simulink model "knee_assist_rev27"  (R2026b)
settings: Solver=ode1  StartTime=0  StopTime=ka_sl.t_end  FixedStep=ka_sl.dt
PostLoadFcn:
  | addpath(fileparts(get_param('knee_assist_rev27', 'FileName')));
InitFcn:
  | addpath(fileparts(get_param('knee_assist_rev27', 'FileName'))); clear sl_ka_logic sl_ka_plant; if ~(exist('ka_sl','var') && exist('ka_p','var') && exist('ka_cfg','var')), ka_simulink_setup; end
undefined symbols (not defined in the file or in its folder): ka_sl, sl_ka_logic, sl_ka_plant
settings Model: Creator=SDP II team  LastModifiedBy=SDP II team
settings DataIOCC: SaveOutput=off  SaveTime=off

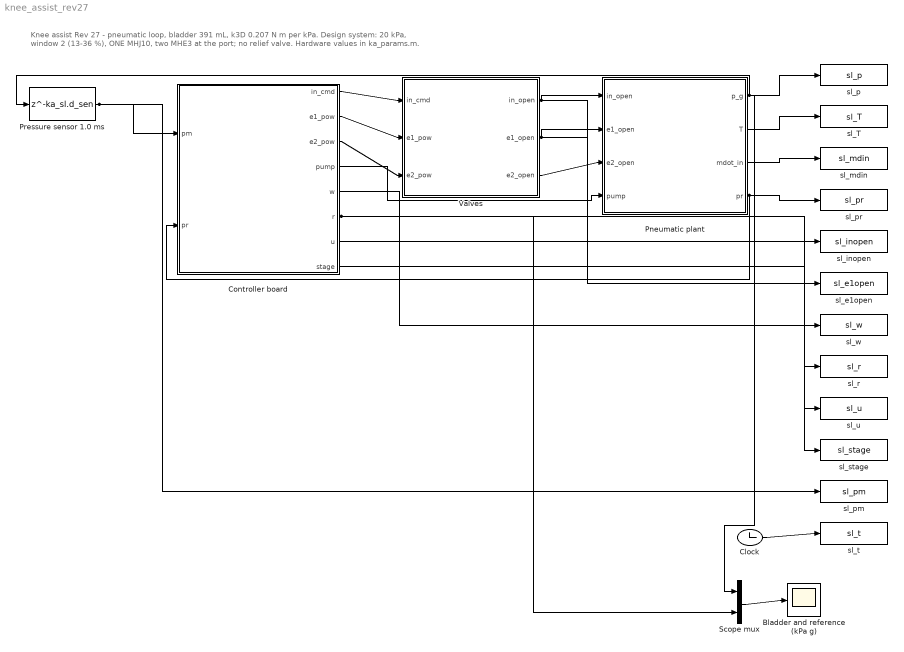
== system knee_assist_rev27 ==
  note: Knee assist Rev 27 - pneumatic loop, bladder 391 mL, k3D 0.207 N m per kPa. Design system: 20 kPa, window 2 (13-36 %), ONE MHJ10, two MHE3 at the port; no relief valve. Hardware values in ka_params.m.
  Bladder and reference (kPa g) : Scope
  Clock : Clock
  Controller board : Subsystem
  Pneumatic plant : Subsystem
  Pressure sensor 1.0 ms : Delay  DelayLength=ka_sl.d_sen  InitialCondition=ka_sl.p0  SampleTime=ka_sl.dt
  Scope mux : Mux  Inputs=2
  Valves : Subsystem
  sl_T : ToWorkspace  VariableName=sl_T  SampleTime=-1
      settings: Decimation=ka_sl.decim
  sl_e1open : ToWorkspace  VariableName=sl_e1open  SampleTime=-1
      settings: Decimation=ka_sl.decim
  sl_inopen : ToWorkspace  VariableName=sl_inopen  SampleTime=-1
      settings: Decimation=ka_sl.decim
  sl_mdin : ToWorkspace  VariableName=sl_mdin  SampleTime=-1
      settings: Decimation=ka_sl.decim
  sl_p : ToWorkspace  VariableName=sl_p  SampleTime=-1
      settings: Decimation=ka_sl.decim
  sl_pm : ToWorkspace  VariableName=sl_pm  SampleTime=-1
      settings: Decimation=ka_sl.decim
  sl_pr : ToWorkspace  VariableName=sl_pr  SampleTime=-1
      settings: Decimation=ka_sl.decim
  sl_r : ToWorkspace  VariableName=sl_r  SampleTime=-1
      settings: Decimation=ka_sl.decim
  sl_stage : ToWorkspace  VariableName=sl_stage  SampleTime=-1
      settings: Decimation=ka_sl.decim
  sl_t : ToWorkspace  VariableName=sl_t  SampleTime=-1
      settings: Decimation=ka_sl.decim
  sl_u : ToWorkspace  VariableName=sl_u  SampleTime=-1
      settings: Decimation=ka_sl.decim
  sl_w : ToWorkspace  VariableName=sl_w  SampleTime=-1
      settings: Decimation=ka_sl.decim
  wires:
  Pneumatic plant/1(p_g) -> Pressure sensor 1.0 ms/1, sl_p/1, Scope mux/1
  Pressure sensor 1.0 ms/1 -> Controller board/1(pm), sl_pm/1
  Pneumatic plant/4(pr) -> Controller board/2(pr), sl_pr/1
  Controller board/1(in_cmd) -> Valves/1(in_cmd)
  Controller board/2(e1_pow) -> Valves/2(e1_pow)
  Controller board/3(e2_pow) -> Valves/3(e2_pow)
  Valves/1(in_open) -> Pneumatic plant/1(in_open), sl_inopen/1
  Valves/2(e1_open) -> Pneumatic plant/2(e1_open), sl_e1open/1
  Valves/3(e2_open) -> Pneumatic plant/3(e2_open)
  Controller board/4(pump) -> Pneumatic plant/4(pump)
  Pneumatic plant/2(T) -> sl_T/1
  Pneumatic plant/3(mdot_in) -> sl_mdin/1
  Controller board/5(w) -> sl_w/1
  Controller board/6(r) -> sl_r/1, Scope mux/2
  Controller board/7(u) -> sl_u/1
  Controller board/8(stage) -> sl_stage/1
  Clock/1 -> sl_t/1
  Scope mux/1 -> Bladder and reference (kPa g)/1

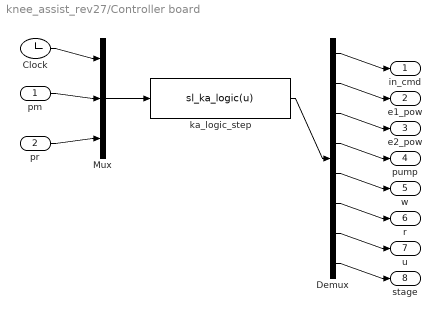
== system knee_assist_rev27/Controller board ==
  pm : Inport
  pr : Inport  Port=2
  Clock : Clock
  Demux : Demux  Outputs=8
  Mux : Mux  Inputs=3
  ka_logic_step : MATLABFcn  MATLABFcn=sl_ka_logic(u)  OutputDimensions=8  SampleTime=ka_sl.dt
  in_cmd : Outport
  e1_pow : Outport  Port=2
  e2_pow : Outport  Port=3
  pump : Outport  Port=4
  w : Outport  Port=5
  r : Outport  Port=6
  u : Outport  Port=7
  stage : Outport  Port=8
  wires:
  Clock/1 -> Mux/1
  pm/1 -> Mux/2
  pr/1 -> Mux/3
  Mux/1 -> ka_logic_step/1
  ka_logic_step/1 -> Demux/1
  Demux/1 -> in_cmd/1
  Demux/2 -> e1_pow/1
  Demux/3 -> e2_pow/1
  Demux/4 -> pump/1
  Demux/5 -> w/1
  Demux/6 -> r/1
  Demux/7 -> u/1
  Demux/8 -> stage/1

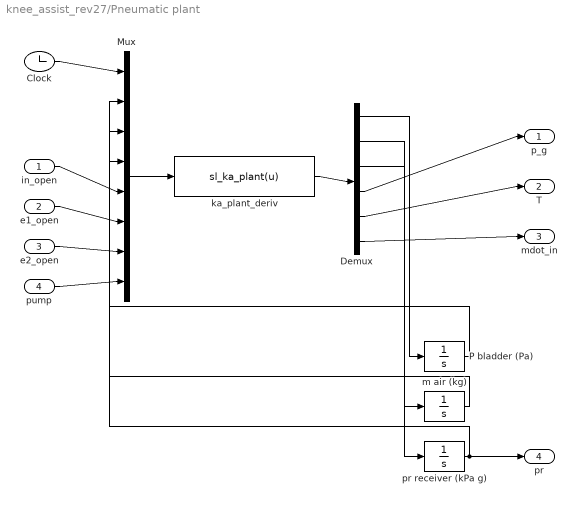
== system knee_assist_rev27/Pneumatic plant ==
  in_open : Inport
  e1_open : Inport  Port=2
  e2_open : Inport  Port=3
  pump : Inport  Port=4
  Clock : Clock
  Demux : Demux  Outputs=6
  Mux : Mux  Inputs=8
  P bladder (Pa) : Integrator  InitialCondition=ka_sl.P0
  ka_plant_deriv : MATLABFcn  MATLABFcn=sl_ka_plant(u)  OutputDimensions=6  SampleTime=0
  m air (kg) : Integrator  InitialCondition=ka_sl.m0
  pr receiver (kPa g) : Integrator  InitialCondition=ka_sl.pr0
  p_g : Outport
  T : Outport  Port=2
  mdot_in : Outport  Port=3
  pr : Outport  Port=4
  wires:
  Clock/1 -> Mux/1
  P bladder (Pa)/1 -> Mux/2
  m air (kg)/1 -> Mux/3
  pr receiver (kPa g)/1 -> Mux/4, pr/1
  in_open/1 -> Mux/5
  e1_open/1 -> Mux/6
  e2_open/1 -> Mux/7
  pump/1 -> Mux/8
  Mux/1 -> ka_plant_deriv/1
  ka_plant_deriv/1 -> Demux/1
  Demux/1 -> P bladder (Pa)/1
  Demux/2 -> m air (kg)/1
  Demux/3 -> pr receiver (kPa g)/1
  Demux/4 -> p_g/1
  Demux/5 -> T/1
  Demux/6 -> mdot_in/1

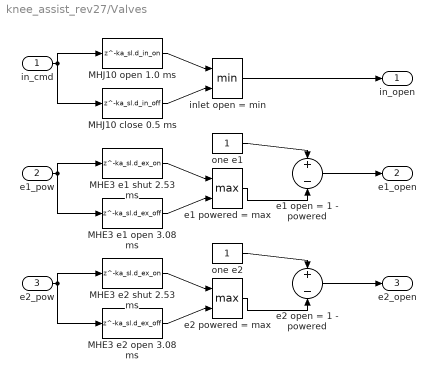
== system knee_assist_rev27/Valves ==
  in_cmd : Inport
  e1_pow : Inport  Port=2
  e2_pow : Inport  Port=3
  MHE3 e1 open 3.08 ms : Delay  DelayLength=ka_sl.d_ex_off  InitialCondition=ka_sl.ex0  SampleTime=ka_sl.dt
  MHE3 e1 shut 2.53 ms : Delay  DelayLength=ka_sl.d_ex_on  InitialCondition=ka_sl.ex0  SampleTime=ka_sl.dt
  MHE3 e2 open 3.08 ms : Delay  DelayLength=ka_sl.d_ex_off  InitialCondition=ka_sl.ex0  SampleTime=ka_sl.dt
  MHE3 e2 shut 2.53 ms : Delay  DelayLength=ka_sl.d_ex_on  InitialCondition=ka_sl.ex0  SampleTime=ka_sl.dt
  MHJ10 close 0.5 ms : Delay  DelayLength=ka_sl.d_in_off  InitialCondition=ka_sl.in0  SampleTime=ka_sl.dt
  MHJ10 open 1.0 ms : Delay  DelayLength=ka_sl.d_in_on  InitialCondition=ka_sl.in0  SampleTime=ka_sl.dt
  e1 open = 1 - powered : Sum  Inputs=+-
  e1 powered = max : MinMax  Function=max  Inputs=2
  e2 open = 1 - powered : Sum  Inputs=+-
  e2 powered = max : MinMax  Function=max  Inputs=2
  inlet open = min : MinMax  Inputs=2
  one e1 : Constant
  one e2 : Constant
  in_open : Outport
  e1_open : Outport  Port=2
  e2_open : Outport  Port=3
  wires:
  in_cmd/1 -> MHJ10 open 1.0 ms/1, MHJ10 close 0.5 ms/1
  MHJ10 open 1.0 ms/1 -> inlet open = min/1
  MHJ10 close 0.5 ms/1 -> inlet open = min/2
  inlet open = min/1 -> in_open/1
  e1_pow/1 -> MHE3 e1 shut 2.53 ms/1, MHE3 e1 open 3.08 ms/1
  MHE3 e1 shut 2.53 ms/1 -> e1 powered = max/1
  MHE3 e1 open 3.08 ms/1 -> e1 powered = max/2
  one e1/1 -> e1 open = 1 - powered/1
  e1 powered = max/1 -> e1 open = 1 - powered/2
  e1 open = 1 - powered/1 -> e1_open/1
  e2_pow/1 -> MHE3 e2 shut 2.53 ms/1, MHE3 e2 open 3.08 ms/1
  MHE3 e2 shut 2.53 ms/1 -> e2 powered = max/1
  MHE3 e2 open 3.08 ms/1 -> e2 powered = max/2
  one e2/1 -> e2 open = 1 - powered/1
  e2 powered = max/1 -> e2 open = 1 - powered/2
  e2 open = 1 - powered/1 -> e2_open/1
